simulink model "discreto"  (R2018a)
settings: Solver=VariableStepAuto  StartTime=0.0  StopTime=12  RelTol=1e-3
undefined symbols (not defined in the file): a, b, c, d, den1, f, num1
settings Model: Creator=Karel  LastModifiedBy=Karel

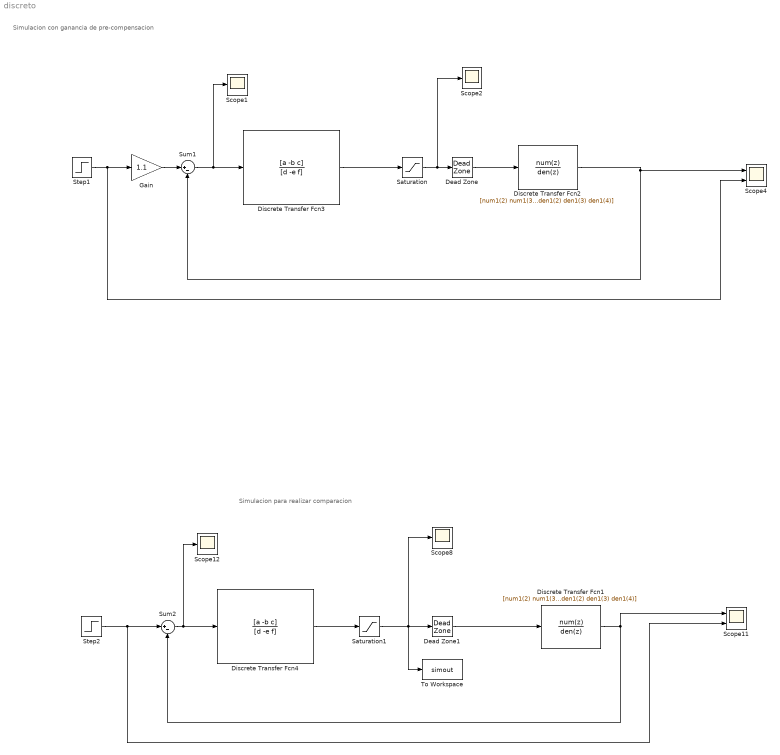
== system discreto ==
  note: Simulacion con ganancia de pre-compensacion
  note: Simulacion para realizar comparacion
  Dead Zone : DeadZone  LowerValue=0  UpperValue=0.2  SaturateOnIntegerOverflow=on
  Dead Zone1 : DeadZone  LowerValue=0  UpperValue=0.2  SaturateOnIntegerOverflow=on
  Discrete Transfer Fcn1 : DiscreteTransferFcn  Numerator=[num1(2) num1(3) num1(4)]  Denominator=[den1(1) den1(2) den1(3) den1(4)]  SampleTime=27e-3
  Discrete Transfer Fcn2 : DiscreteTransferFcn  Numerator=[num1(2) num1(3) num1(4)]  Denominator=[den1(1) den1(2) den1(3) den1(4)]  SampleTime=27e-3
  Discrete Transfer Fcn3 : DiscreteTransferFcn  Numerator=[a -b c]  Denominator=[d -e f]  SampleTime=27e-03
  Discrete Transfer Fcn4 : DiscreteTransferFcn  Numerator=[a -b c]  Denominator=[d -e f]  SampleTime=27e-03
  Gain : Gain  Gain=1.1
  Saturation : Saturate  UpperLimit=10  LowerLimit=0
  Saturation1 : Saturate  UpperLimit=10  LowerLimit=0
  Scope{1..2,8,12} (4 alike) : Scope
  Scope11 : Scope  NumInputPorts=2
  Scope4 : Scope  NumInputPorts=2
  Step1 : Step  Time=0  After=10  SampleTime=0
  Step2 : Step  Time=5.27  After=10  SampleTime=0
  Sum1 : Sum  Inputs=|+-
  Sum2 : Sum  Inputs=|+-
  To Workspace : ToWorkspace  VariableName=simout  SaveFormat=Structure With Time  SampleTime=1e-3
  wires:
  Discrete Transfer Fcn3/1 -> Saturation/1
  Discrete Transfer Fcn2/1 -> Sum1/2, Scope4/1
  Dead Zone/1 -> Discrete Transfer Fcn2/1
  Step1/1 -> Scope4/2, Gain/1
  Gain/1 -> Sum1/1
  Step2/1 -> Sum2/1, Scope11/2
  Dead Zone1/1 -> Discrete Transfer Fcn1/1
  Sum2/1 -> Scope12/1, Discrete Transfer Fcn4/1
  Discrete Transfer Fcn1/1 -> Scope11/1, Sum2/2
  Discrete Transfer Fcn4/1 -> Saturation1/1
  Saturation1/1 -> To Workspace/1, Scope8/1, Dead Zone1/1
  Saturation/1 -> Scope2/1, Dead Zone/1
  Sum1/1 -> Scope1/1, Discrete Transfer Fcn3/1
